simulink model "structure_contact"  (R2026b)
settings: Solver=VariableStepAuto
undefined symbols (not defined in the file or in its folder): P
libraries: sharedutil x1
settings Model: Creator=aomar  LastModifiedBy=aomar

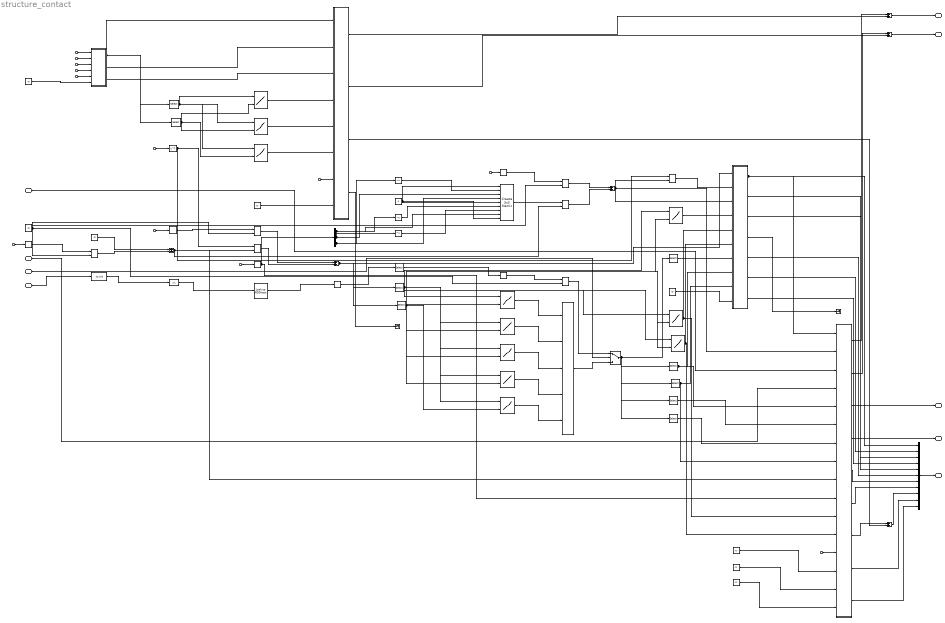
== system structure_contact ==
  body_Xe : Inport  PortName=body  Element=Xe
  body_Xe_2 : Inport  PortName=body  Element=Xe
  body_Vb : Inport  PortName=body  Element=Vb
  body_Vb_2 : Inport  PortName=body  Element=Vb
  body_omega : Inport  PortName=body  Element=omega
  body_omega_2 : Inport  PortName=body  Element=omega
  body_r_cg : Inport  PortName=body  Element=r_cg
  body_r_cg_2 : Inport  PortName=body  Element=r_cg
  body_DCM_be : Inport  PortName=body  Element=DCM_be
  body_DCM_be_2 : Inport  PortName=body  Element=DCM_be
  body_DCM_be_3 : Inport  PortName=body  Element=DCM_be
  body_DCM_be_4 : Inport  PortName=body  Element=DCM_be
  s : Inport  Port=2
  vB_d : Inport  Port=3
  use_soil : Inport  Port=4
  soil_id : Inport  Port=5
  C_nb : Math  Operator=transpose
  Cnb_rj : Product  Inputs=**  Multiplication=Matrix(*)
  Contact_Diag : BusCreator  Inputs=11
  E_g : Selector  NumberOfDimensions=2  InputPortWidth=3  IndexOptions=Index vector (dialog),Select all  Indices=2,1  OutputSizes=1
  E_j : Selector  NumberOfDimensions=2  InputPortWidth=3  IndexOptions=Index vector (dialog),Select all  Indices=2,1  OutputSizes=1
  F_c_sum : Sum
  H : Lookup_n-D  BreakpointsForDimension1=P.world.terrain.xE  BreakpointsForDimension2=P.world.terrain.yN  IndexSearchMethod=Evenly spaced points  Table=P.world.terrain.H  ExtrapMethod=Clip  InternalRulePriority=Speed  RndMeth=Simplest
      settings: InputPortMap=u0,u1
  H_g : Lookup_n-D  BreakpointsForDimension1=P.world.terrain.xE  BreakpointsForDimension2=P.world.terrain.yN  IndexSearchMethod=Evenly spaced points  Table=P.world.terrain.H  ExtrapMethod=Clip  InternalRulePriority=Speed  RndMeth=Simplest
      settings: InputPortMap=u0,u1
  K : Selector  NumberOfDimensions=2  InputPortWidth=3  IndexOptions=Index vector (dialog),Select all  Indices=2,1  OutputSizes=1
  K_map : Lookup_n-D  BreakpointsForDimension1=P.world.terrain.xE  BreakpointsForDimension2=P.world.terrain.yN  IndexSearchMethod=Evenly spaced points  Table=P.world.soil.K  ExtrapMethod=Clip  InternalRulePriority=Speed  RndMeth=Simplest
      settings: InputPortMap=u0,u1
  MF_A_trackContactNormal : MATLAB Function  TreatAsAtomicUnit=on
  MF_B_trackPlanarForces : MATLAB Function  TreatAsAtomicUnit=on
  MF_C1_gaugeWheelPoints : MATLAB Function  TreatAsAtomicUnit=on
  MF_C2_gaugeWheelContact : MATLAB Function  TreatAsAtomicUnit=on
  M_c_sum : Sum
  N_g : Selector  NumberOfDimensions=2  InputPortWidth=3  IndexOptions=Index vector (dialog),Select all  Indices=1,1  OutputSizes=1
  N_j : Selector  NumberOfDimensions=2  InputPortWidth=3  IndexOptions=Index vector (dialog),Select all  Indices=1,1  OutputSizes=1
  Omega_hat : sharedutil/Create 3x3 Matrix  aMode=aMode
      settings: LibrarySourceBlock=aerolibutil/Create 3x3 Matrix
  Ones : Constant  Value=ones(1,2*P.structure.track.Nc)  VectorParams1D=off
  P_diss_sum : Sum
  Pn : Sum
  Rc_R : Constant  Value=P.structure.contact.Rc_R  VectorParams1D=off
  Rcg_rep : Product  Inputs=**  Multiplication=Matrix(*)
  Rg_R : Constant  Value=P.structure.contact.gw.R  VectorParams1D=off
  Soil_col : Reshape  OutputDimensionality=Column vector (2-D)
  Soil_map : Concatenate  NumInputs=5  Mode=Multidimensional array
  Soil_props : Selector  InputPortWidth=6  IndexOptions=Index vector (dialog)  Indices=2:6  OutputSizes=1
  Soil_rep : Product  Inputs=**  Multiplication=Matrix(*)
  Soil_row : Reshape
  Soil_sw : Switch  Criteria=u2 ~= 0  SaturateOnIntegerOverflow=off  InputSameDT=off
  Soil_table : LookupNDDirect  InputsSelectThisObjectFromTable=Vector  Table=P.world.soilTable'  DiagnosticForOutOfRangeInput=None
  Term_K_trk : Terminator
  Term_N_gw : Terminator
  Vb_col : Reshape  OutputDimensionality=Column vector (2-D)
  Vb_pt : Sum
  Vb_rep : Product  Inputs=**  Multiplication=Matrix(*)
  Vn : Product  Inputs=**  Multiplication=Matrix(*)
  Wxr : Product  Inputs=**  Multiplication=Matrix(*)
  Xe_col : Reshape  OutputDimensionality=Column vector (2-D)
  Xe_rep : Product  Inputs=**  Multiplication=Matrix(*)
  Zero : Constant  Value=0  VectorParams1D=off
  dHdE : Lookup_n-D  BreakpointsForDimension1=P.world.terrain.xE  BreakpointsForDimension2=P.world.terrain.yN  IndexSearchMethod=Evenly spaced points  Table=P.world.terrain.dHdE  ExtrapMethod=Clip  InternalRulePriority=Speed  RndMeth=Simplest
      settings: InputPortMap=u0,u1
  dHdE_g : Lookup_n-D  BreakpointsForDimension1=P.world.terrain.xE  BreakpointsForDimension2=P.world.terrain.yN  IndexSearchMethod=Evenly spaced points  Table=P.world.terrain.dHdE  ExtrapMethod=Clip  InternalRulePriority=Speed  RndMeth=Simplest
      settings: InputPortMap=u0,u1
  dHdN : Lookup_n-D  BreakpointsForDimension1=P.world.terrain.xE  BreakpointsForDimension2=P.world.terrain.yN  IndexSearchMethod=Evenly spaced points  Table=P.world.terrain.dHdN  ExtrapMethod=Clip  InternalRulePriority=Speed  RndMeth=Simplest
      settings: InputPortMap=u0,u1
  dHdN_g : Lookup_n-D  BreakpointsForDimension1=P.world.terrain.xE  BreakpointsForDimension2=P.world.terrain.yN  IndexSearchMethod=Evenly spaced points  Table=P.world.terrain.dHdN  ExtrapMethod=Clip  InternalRulePriority=Speed  RndMeth=Simplest
      settings: InputPortMap=u0,u1
  fR : Selector  NumberOfDimensions=2  InputPortWidth=3  IndexOptions=Index vector (dialog),Select all  Indices=4,1  OutputSizes=1
  fRoll_map : Lookup_n-D  BreakpointsForDimension1=P.world.terrain.xE  BreakpointsForDimension2=P.world.terrain.yN  IndexSearchMethod=Evenly spaced points  Table=P.world.soil.fRoll  ExtrapMethod=Clip  InternalRulePriority=Speed  RndMeth=Simplest
      settings: InputPortMap=u0,u1
  gG : Constant  Value=P.structure.track.gG  VectorParams1D=off
  gS : Constant  Value=P.structure.track.gS  VectorParams1D=off
  kS : Selector  NumberOfDimensions=2  InputPortWidth=3  IndexOptions=Index vector (dialog),Select all  Indices=5,1  OutputSizes=1
  kScale_map : Lookup_n-D  BreakpointsForDimension1=P.world.terrain.xE  BreakpointsForDimension2=P.world.terrain.yN  IndexSearchMethod=Evenly spaced points  Table=P.world.soil.kScale  ExtrapMethod=Clip  InternalRulePriority=Speed  RndMeth=Simplest
      settings: InputPortMap=u0,u1
  muLat : Selector  NumberOfDimensions=2  InputPortWidth=3  IndexOptions=Index vector (dialog),Select all  Indices=3,1  OutputSizes=1
  muLat_map : Lookup_n-D  BreakpointsForDimension1=P.world.terrain.xE  BreakpointsForDimension2=P.world.terrain.yN  IndexSearchMethod=Evenly spaced points  Table=P.world.soil.muLat  ExtrapMethod=Clip  InternalRulePriority=Speed  RndMeth=Simplest
      settings: InputPortMap=u0,u1
  muP : Selector  NumberOfDimensions=2  InputPortWidth=3  IndexOptions=Index vector (dialog),Select all  Indices=1,1  OutputSizes=1
  muPeak_map : Lookup_n-D  BreakpointsForDimension1=P.world.terrain.xE  BreakpointsForDimension2=P.world.terrain.yN  IndexSearchMethod=Evenly spaced points  Table=P.world.soil.muPeak  ExtrapMethod=Clip  InternalRulePriority=Speed  RndMeth=Simplest
      settings: InputPortMap=u0,u1
  neg_p : UnaryMinus
  neg_q : UnaryMinus
  neg_r : UnaryMinus
  pqr : Demux  Outputs=3
  prmC : Constant  Value=[P.structure.contact.kc; P.structure.contact.cc]  VectorParams1D=off
  prmG : Constant  Value=[P.structure.contact.gw.on; P.structure.contact.gw.k; P.structure.contact.gw.c]  VectorParams1D=off
  prmT : Constant  Value=[P.structure.track.ell; P.structure.track.tau_d; P.structure.track.vEpsRR; P.structure.track.B; P.structure.track.chi_rmin]  VectorParams1D=off
  r_j : Sum  Inputs=+-
  rcg_col : Reshape  OutputDimensionality=Column vector (2-D)
  soil_dbl : DataTypeConversion  OutDataTypeStr=double  SaturateOnIntegerOverflow=off  RndMeth=Floor
  soil_idx0 : Bias  Bias=-1  SaturateOnIntegerOverflow=off
  w_col : Reshape  OutputDimensionality=Column vector (2-D)
  F_c : Outport
  M_c : Outport  Port=2
  sDot : Outport  Port=3
  Fx_pt : Outport  Port=4
  cdiag : Outport  Port=5
  wires:
  body_r_cg/1 -> rcg_col/1  "r_cg"
  Rg_R/1 -> MF_C1_gaugeWheelPoints/6(Rg)  "Rg_R"
  s/1 -> MF_B_trackPlanarForces/3(s)  "s"
  Ones/1 -> Soil_rep/2, Vb_rep/2, Rcg_rep/2, Xe_rep/2  "ones"
  rcg_col/1 -> Rcg_rep/1  "rcg_col"
  vB_d/1 -> MF_B_trackPlanarForces/4(vB)  "vB_d"
  use_soil/1 -> Soil_sw/2  "use_soil"
  soil_id/1 -> soil_dbl/1  "soil_id"
  body_Xe_2/1 -> MF_C1_gaugeWheelPoints/1(Xe)  "Xe"
  body_DCM_be_3/1 -> MF_C1_gaugeWheelPoints/2(DCM_be)  "DCM_be"
  body_Vb_2/1 -> MF_C1_gaugeWheelPoints/3(Vb)  "Vb"
  body_omega_2/1 -> MF_C1_gaugeWheelPoints/4(omega)  "omega"
  body_r_cg_2/1 -> MF_C1_gaugeWheelPoints/5(rcg)  "r_cg"
  Rc_R/1 -> r_j/1  "Rc_R"
  Rcg_rep/1 -> r_j/2  "Rcg_rep"
  MF_C1_gaugeWheelPoints/1(Pn_g) -> N_g/1, E_g/1, MF_C2_gaugeWheelContact/1(Pn_g)  "Pn_g"
  MF_C1_gaugeWheelPoints/2(Vn_g) -> MF_C2_gaugeWheelContact/2(Vn_g)  "Vn_g"
  MF_C1_gaugeWheelPoints/3(r_g) -> MF_C2_gaugeWheelContact/3(r_g)  "r_g"
  soil_dbl/1 -> soil_idx0/1  "soil_dbl"
  body_DCM_be/1 -> C_nb/1  "DCM_be"
  body_Xe/1 -> Xe_col/1  "Xe"
  r_j/1 -> MF_B_trackPlanarForces/9(Rcg), Wxr/2, Cnb_rj/2  "r_j"
  C_nb/1 -> Cnb_rj/1, Vn/1  "C_nb"
  Xe_col/1 -> Xe_rep/1  "Xe_col"
  E_g/1 -> dHdN_g/1, dHdE_g/1, H_g/1  "E_g"
  soil_idx0/1 -> Soil_table/1  "soil_index0"
  N_g/1 -> dHdN_g/2, H_g/2, dHdE_g/2  "N_g"
  body_omega/1 -> w_col/1  "omega"
  prmG/1 -> MF_C2_gaugeWheelContact/8(prmG)  "prmG"
  Xe_rep/1 -> Pn/1  "Xe_rep"
  Cnb_rj/1 -> Pn/2  "Cnb_rj"
  w_col/1 -> MF_B_trackPlanarForces/10(omega), pqr/1  "w_col"
  H_g/1 -> MF_C2_gaugeWheelContact/4(h)  "h_g"
  dHdE_g/1 -> MF_C2_gaugeWheelContact/5(hE)  "hE_g"
  dHdN_g/1 -> MF_C2_gaugeWheelContact/6(hN)  "hN_g"
  Soil_table/1 -> Soil_row/1  "soil_row"
  body_DCM_be_4/1 -> MF_C2_gaugeWheelContact/7(DCM_be)  "DCM_be"
  pqr/1 -> Omega_hat/8, neg_p/1  "p"
  pqr/2 -> Omega_hat/3, neg_q/1  "q"
  pqr/3 -> neg_r/1, Omega_hat/4  "r"
  Pn/1 -> MF_A_trackContactNormal/1(Pn), N_j/1, E_j/1  "Pn"
  Soil_row/1 -> Soil_props/1  "Soil_row"
  MF_C2_gaugeWheelContact/1(F_g) -> F_c_sum/2  "F_gw"
  MF_C2_gaugeWheelContact/2(M_g) -> M_c_sum/2  "M_gw"
  MF_C2_gaugeWheelContact/3(P_g) -> P_diss_sum/2  "P_gw"
  MF_C2_gaugeWheelContact/4(N_g) -> Term_N_gw/1  "N_gw"
  neg_r/1 -> Omega_hat/2  "neg_r"
  Zero/1 -> Omega_hat/9, Omega_hat/1, Omega_hat/5  "Zero"
  neg_p/1 -> Omega_hat/6  "neg_p"
  neg_q/1 -> Omega_hat/7  "neg_q"
  Soil_props/1 -> Soil_col/1  "soil_props5"
  E_j/1 -> kScale_map/1, fRoll_map/1, H/1, muLat_map/1, dHdN/1, K_map/1, dHdE/1, muPeak_map/1  "E_j"
  N_j/1 -> kScale_map/2, H/2, fRoll_map/2, muLat_map/2, dHdN/2, K_map/2, dHdE/2, muPeak_map/2  "N_j"
  body_Vb/1 -> Vb_col/1  "Vb"
  Vb_col/1 -> Vb_rep/1  "Vb_col"
  Soil_col/1 -> Soil_rep/1  "Soil_col"
  Omega_hat/1 -> Wxr/1  "Omega_hat"
  muPeak_map/1 -> Soil_map/1  "muPeak"
  K_map/1 -> Soil_map/2  "K"
  muLat_map/1 -> Soil_map/3  "muLat"
  fRoll_map/1 -> Soil_map/4  "fRoll"
  kScale_map/1 -> Soil_map/5  "kScale"
  Vb_rep/1 -> Vb_pt/1  "Vb_rep"
  Wxr/1 -> Vb_pt/2  "Wxr"
  Soil_rep/1 -> Soil_sw/1  "soil_ovr"
  Soil_map/1 -> Soil_sw/3  "soil_map"
  Vb_pt/1 -> MF_B_trackPlanarForces/2(Vb_pt), MF_A_trackContactNormal/3(Vb_pt), Vn/2  "Vb_pt"
  Soil_sw/1 -> kS/1, fR/1, muLat/1, K/1, muP/1  "soil_props"
  Vn/1 -> MF_A_trackContactNormal/2(Vn)  "Vn"
  prmC/1 -> MF_A_trackContactNormal/10(prmC)  "prmC"
  kS/1 -> MF_A_trackContactNormal/7(kS)  "kS"
  muP/1 -> MF_A_trackContactNormal/8(muP), MF_B_trackPlanarForces/5(muP)  "muP"
  muLat/1 -> MF_B_trackPlanarForces/6(muLat)  "muLat"
  fR/1 -> MF_B_trackPlanarForces/7(fR)  "fR"
  K/1 -> MF_A_trackContactNormal/9(K), MF_B_trackPlanarForces/8(K)  "K"
  H/1 -> MF_A_trackContactNormal/4(h)  "h"
  prmT/1 -> MF_B_trackPlanarForces/14(prmT)  "prmT"
  gS/1 -> MF_B_trackPlanarForces/15(gS)  "gS"
  gG/1 -> MF_B_trackPlanarForces/16(gG)  "gG"
  MF_A_trackContactNormal/1(N_pt) -> Contact_Diag/1, MF_B_trackPlanarForces/1(N_pt)  "N_pt"
  MF_A_trackContactNormal/2(N_trk) -> Contact_Diag/3  "N_trk"
  MF_A_trackContactNormal/3(muP_trk) -> Contact_Diag/5  "muP_trk"
  MF_A_trackContactNormal/4(K_trk) -> Term_K_trk/1  "K_trk"
  MF_A_trackContactNormal/5(vG_trk) -> Contact_Diag/6  "vG_trk"
  MF_A_trackContactNormal/6(pen_pt) -> Contact_Diag/2  "pen_pt"
  MF_A_trackContactNormal/7(sink_trk) -> Contact_Diag/4  "sink_trk"
  body_DCM_be_2/1 -> MF_B_trackPlanarForces/13(DCM_be)  "DCM_be"
  MF_B_trackPlanarForces/1(F_c) -> F_c_sum/1  "F_c_trk"
  MF_B_trackPlanarForces/2(M_c) -> M_c_sum/1  "M_c_trk"
  MF_B_trackPlanarForces/3(sDot) -> sDot/1  "sDot"
  MF_B_trackPlanarForces/4(Fx_pt) -> Fx_pt/1  "Fx_pt"
  MF_B_trackPlanarForces/5(Fy_trk) -> Contact_Diag/7  "Fy_trk"
  MF_B_trackPlanarForces/6(M_turn) -> Contact_Diag/8  "M_turn"
  MF_B_trackPlanarForces/7(P_diss) -> P_diss_sum/1  "P_diss_trk"
  MF_B_trackPlanarForces/8(chi_eff) -> Contact_Diag/10  "chi_eff"
  MF_B_trackPlanarForces/9(s_trk) -> Contact_Diag/11  "s_trk"
  F_c_sum/1 -> F_c/1  "F_c"
  M_c_sum/1 -> M_c/1  "M_c"
  P_diss_sum/1 -> Contact_Diag/9  "P_diss"
  Contact_Diag/1 -> cdiag/1  "cdiag"
  dHdE/1 -> MF_B_trackPlanarForces/11(hE), MF_A_trackContactNormal/5(hE)  "hE"
  dHdN/1 -> MF_B_trackPlanarForces/12(hN), MF_A_trackContactNormal/6(hN)  "hN"

== matlab function structure_contact/MF_B_trackPlanarForces ==
  settings: description=MF-B: isotropic 2-D shear law, rolling resistance, contact wrench (structure_planar_forces.m); prmT = [ell; tau_d; vEpsRR; B; chi_rmin], gS / gG of P.structure.track
  data: N_pt input; F_c output; Vb_pt input; s input; vB input; muP input; muLat input; fR input; K input; Rcg input; omega input; hE input; hN input; DCM_be input; prmT input; gS input; gG input; M_c output; sDot output; Fx_pt output; Fy_trk output; M_turn output; P_diss output; chi_eff output; s_trk output
function [F_c, M_c, sDot, Fx_pt, Fy_trk, M_turn, P_diss, chi_eff, s_trk] = trackPlanarForces(N_pt, Vb_pt, s, vB, muP, muLat, fR, K, Rcg, omega, hE, hN, DCM_be, prmT, gS, gG)
%#codegen
[F_c, M_c, sDot, Fx_pt, Fy_trk, M_turn, P_diss, chi_eff, s_trk] = structure_planar_forces(N_pt, Vb_pt, s, vB, muP, muLat, fR, K, Rcg, omega, hE, hN, DCM_be, struct('ell', prmT(1), 'tau_d', prmT(2), 'vEpsRR', prmT(3), 'B', prmT(4), 'chi_rmin', prmT(5), 'gS', gS, 'gG', gG));
end

% ---- verbatim copy of subsystems/structure/structure_planar_forces.m (generated by build_structure, do not edit here) ----
function [F_c, M_c, sDot, Fx_pt, Fy_trk, M_turn, P_diss, chi_eff, s_trk] = structure_planar_forces(N_pt, Vb_pt, s, vB, muP, muLat, fR, K, Rcg, omega, hE, hN, DCM_be, prm)
%STRUCTURE_PLANAR_FORCES  MF-B trackPlanarForces: per-point ISOTROPIC 2-D Dahl/Janosi shear (revision B, D39),
%   rolling resistance and the contact wrench (docs/specs/structure.md 2.5 / 2.6 / 4.2; owner structure, T03).
%#codegen
%
%   Inputs  N_pt [M x 1] normal forces (MF-A), Vb_pt [3 x M] point velocities in body axes (FRD),
%           s [2M x 1] shear states [s_x(1:M); s_y(1:M)] (Integrator, structure_track_shear),
%           vB [2 x 1] belt speeds [L; R] DELAYED by one 1 ms sample (D36 loop breaker),
%           muP, muLat, fR, K [1 x M] soil properties at the points, Rcg [3 x M] lever arms w.r.t. the CG (FRD),
%           omega [3 x 1] body rates (FRD), hE, hN [1 x M] terrain gradients at the points, DCM_be [3 x 3] NED->body,
%           prm = struct with the P.structure.track fields ell, tau_d, vEpsRR, gS, gG, B, chi_rmin (Nc = numel(N_pt)/2)
%   Per point j of track i:
%     v_slip = [v_b,i - v_x,j; -v_y,j]                       (belt minus ground)
%     ds/dt  = (v_slip - |v_slip| s)/K_j - (|v_b,i|/ell) s     (2-vector, |s| <= 1)
%     mu_j   = mu_p mu_lat |s| / sqrt((mu_lat s_x)^2 + (mu_p s_y)^2)   (friction ellipse along s; mu_p for |s| < 1e-6)
%     F_j    = sat_|.|( mu_j N_j [g(|s|) s/|s| + tau_d ds/dt], mu_j N_j ),  g = table prm.gS / prm.gG
%     F_rr,j = -f_r,j N_j tanh(v_x,j / vEpsRR)                (rolling resistance, body only)
%     F_c,j  = [F_x,j + F_rr,j; F_y,j; 0] + N_j n_j  applied at r_j, n_j = DCM_be [-hN; -hE; -1]/sqrt(1+hE^2+hN^2)
%              (normal force along the local terrain normal, expressed in body axes; T03 refinement of spec 2.6,
%              which applied it along -z_b: removes the spurious N sin(pitch) force of the static compliance pitch)
%   Outputs F_c, M_c [3 x 1] contact wrench about the CG (FRD), sDot [2M x 1], Fx_pt [M x 1] shear traction per
%           point (sum per track = sprocket belt load), Fy_trk [2 x 1] lateral shear force per track (FRD),
%           M_turn lateral-shear yaw moment sum(x_j F_y,j) (FRD z), P_diss = sum_i F_x,i v_b,i - sum_j F_c,j . v_j
%           (contact dissipation incl. shear slip, rolling resistance and normal damping), chi_eff =
%           (v_bR - v_bL)/(B r_FLU) (NaN for |r| < chi_rmin), s_trk [2 x 1] N-weighted mean s_x per track
M  = numel(N_pt);              % 2*Nc points (compile-time constant from the input dimension)
Nc = M/2;
F_pt = zeros(3, M);
sDot = zeros(2*M, 1);
Fx_pt = zeros(M, 1);
Fy_pt = zeros(M, 1);
gS = prm.gS;  gG = prm.gG;
for j = 1:M
    if j <= Nc, i = 1; else, i = 2; end
    vb  = vB(i);
    vx  = Vb_pt(1, j);  vy = Vb_pt(2, j);
    vsx = vb - vx;      vsy = -vy;
    vsn = sqrt(vsx*vsx + vsy*vsy);
    sx  = s(j);         sy = s(M + j);
    Kj  = max(K(j), 1e-6);
    rl  = abs(vb)/prm.ell;
    dsx = (vsx - vsn*sx)/Kj - rl*sx;
    dsy = (vsy - vsn*sy)/Kj - rl*sy;
    sDot(j) = dsx;  sDot(M + j) = dsy;
    sn  = sqrt(sx*sx + sy*sy);
    if sn < 1e-6
        mu = muP(j);  gx = 0;  gy = 0;
    else
        mu = muP(j)*muLat(j)*sn/sqrt((muLat(j)*sx)^2 + (muP(j)*sy)^2);
        gv = local_g(min(sn, 1), gS, gG);
        gx = gv*sx/sn;  gy = gv*sy/sn;
    end
    cap = mu*N_pt(j);
    fx  = cap*(gx + prm.tau_d*dsx);
    fy  = cap*(gy + prm.tau_d*dsy);
    fm  = sqrt(fx*fx + fy*fy);
    if fm > cap && fm > 0
        fx = fx*cap/fm;  fy = fy*cap/fm;
    end
    frr = -fR(j)*N_pt(j)*tanh(vx/prm.vEpsRR);
    nz  = 1/sqrt(1 + hE(j)^2 + hN(j)^2);
    nN  = -hN(j)*nz;  nE = -hE(j)*nz;  nD = -nz;            % upward terrain normal (NED)
    Fx_pt(j) = fx;  Fy_pt(j) = fy;
    F_pt(1, j) = fx + frr + N_pt(j)*(DCM_be(1,1)*nN + DCM_be(1,2)*nE + DCM_be(1,3)*nD);
    F_pt(2, j) = fy       + N_pt(j)*(DCM_be(2,1)*nN + DCM_be(2,2)*nE + DCM_be(2,3)*nD);
    F_pt(3, j) =            N_pt(j)*(DCM_be(3,1)*nN + DCM_be(3,2)*nE + DCM_be(3,3)*nD);
end
F_c = zeros(3, 1);  M_c = zeros(3, 1);
P_body = 0;  M_turn = 0;
Fy_trk = zeros(2, 1);  Fx_trk = zeros(2, 1);
for j = 1:M
    if j <= Nc, i = 1; else, i = 2; end
    f = F_pt(:, j);  r = Rcg(:, j);
    F_c = F_c + f;
    M_c = M_c + [r(2)*f(3) - r(3)*f(2); r(3)*f(1) - r(1)*f(3); r(1)*f(2) - r(2)*f(1)];
    P_body = P_body + f(1)*Vb_pt(1, j) + f(2)*Vb_pt(2, j) + f(3)*Vb_pt(3, j);
    M_turn = M_turn + r(1)*Fy_pt(j);
    Fy_trk(i) = Fy_trk(i) + Fy_pt(j);
    Fx_trk(i) = Fx_trk(i) + Fx_pt(j);
end
P_diss = Fx_trk(1)*vB(1) + Fx_trk(2)*vB(2) - P_body;
rF = -omega(3);                                  % yaw rate FLU (+ = left turn)
if abs(rF) < prm.chi_rmin
    chi_eff = NaN;
else
    chi_eff = (vB(2) - vB(1))/(prm.B*rF);
end
s_trk = zeros(2, 1);
for i = 1:2
    i0 = (i - 1)*Nc;
    sN = 0;  a = 0;  b = 0;
    for k = 1:Nc
        sN = sN + N_pt(i0 + k);
        a  = a + N_pt(i0 + k)*s(i0 + k);
        b  = b + s(i0 + k)/Nc;
    end
    if sN < 1
        s_trk(i) = b;
    else
        s_trk(i) = a/sN;
    end
end
end

% -------------------------------------------------------------------------------------------
function y = local_g(x, gS, gG)
% codegen-safe linear interpolation of the lumped Janosi table g(s) (same data as P.structure.track.gS/gG)
n = numel(gS);
if x <= gS(1)
    y = gG(1);
elseif x >= gS(n)
    y = gG(n);
else
    k = 1;
    while k < n - 1 && gS(k + 1) < x
        k = k + 1;
    end
    y = gG(k) + (gG(k + 1) - gG(k))*(x - gS(k))/(gS(k + 1) - gS(k));
end
end

== matlab function structure_contact/MF_A_trackContactNormal ==
  settings: description=MF-A: compliant normal contact of the 14 track points (structure_contact_normal.m); prmC = [kc; cc] of P.structure.contact
  data: Pn input; N_pt output; Vn input; Vb_pt input; h input; hE input; hN input; kS input; muP input; K input; prmC input; N_trk output; muP_trk output; K_trk output; vG_trk output; pen_pt output; sink_trk output
function [N_pt, N_trk, muP_trk, K_trk, vG_trk, pen_pt, sink_trk] = trackContactNormal(Pn, Vn, Vb_pt, h, hE, hN, kS, muP, K, prmC)
%#codegen
[N_pt, N_trk, muP_trk, K_trk, vG_trk, pen_pt, sink_trk] = structure_contact_normal(Pn, Vn, Vb_pt, h, hE, hN, kS, muP, K, struct('kc', prmC(1), 'cc', prmC(2)));
end

% ---- verbatim copy of subsystems/structure/structure_contact_normal.m (generated by build_structure, do not edit here) ----
function [N_pt, N_trk, muP_trk, K_trk, vG_trk, pen_pt, sink_trk] = structure_contact_normal(Pn, Vn, Vb_pt, h, hE, hN, kS, muP, K, prm)
%STRUCTURE_CONTACT_NORMAL  MF-A trackContactNormal: compliant normal contact of the 2 x Nc track points
%   (docs/specs/structure.md 2.4 / 4.1; owner structure, build task T03).
%#codegen
%
%   Inputs  Pn, Vn [3 x M] contact-point positions / velocities in NED (M = 2*prm.Nc, 1..Nc left, Nc+1..M right)
%           Vb_pt  [3 x M] contact-point velocities in body axes (FRD)
%           h, hE, hN, kS, muP, K [1 x M] terrain height (up), gradients dH/dE, dH/dN, stiffness scale,
%                  peak traction coefficient and shear modulus at the points (2-D Lookup Tables)
%           prm    struct with the P.structure.contact fields kc, cc (Nc = numel(h)/2 from the inputs)
%   Outputs N_pt [M x 1] normal force (>= 0), N_trk [2 x 1], muP_trk / K_trk [2 x 1] N-weighted means
%           (plain means while N_trk < 1 N), vG_trk [2 x 1] mean body-x ground speed of the track points,
%           pen_pt [M x 1] penetration (> 0 below the surface), sink_trk [2 x 1] N-weighted mean penetration
%
%   pen_j  = (D_j + h_j) n_z,  pen'_j = (vD_j + hE vE_j + hN vN_j) n_z,  n_z = 1/sqrt(1 + hE^2 + hN^2)
%   N_j    = [pen_j > 0] max(0, kc kS_j pen_j + cc sqrt(kS_j) pen'_j)
M  = numel(h);                 % 2*Nc points (compile-time constant from the input dimension)
Nc = M/2;
N_pt = zeros(M, 1);  pen_pt = zeros(M, 1);
N_trk = zeros(2, 1); muP_trk = zeros(2, 1); K_trk = zeros(2, 1); vG_trk = zeros(2, 1); sink_trk = zeros(2, 1);
for j = 1:M
    nz   = 1/sqrt(1 + hE(j)^2 + hN(j)^2);
    pen  = (Pn(3,j) + h(j))*nz;
    penD = (Vn(3,j) + hE(j)*Vn(2,j) + hN(j)*Vn(1,j))*nz;
    pen_pt(j) = pen;
    if pen > 0
        N_pt(j) = max(0, prm.kc*kS(j)*pen + prm.cc*sqrt(kS(j))*penD);
    end
end
for i = 1:2
    i0 = (i - 1)*Nc;
    sN = 0;
    for k = 1:Nc
        sN = sN + N_pt(i0 + k);
    end
    N_trk(i) = sN;
    a = 0; b = 0; c = 0; v = 0;
    for k = 1:Nc
        if sN < 1
            w = 1/Nc;
        else
            w = N_pt(i0 + k)/sN;
        end
        a = a + w*muP(i0 + k);
        b = b + w*K(i0 + k);
        c = c + w*pen_pt(i0 + k);
        v = v + Vb_pt(1, i0 + k)/Nc;
    end
    muP_trk(i) = a;  K_trk(i) = b;  sink_trk(i) = c;  vG_trk(i) = v;
end
end

== matlab function structure_contact/MF_C1_gaugeWheelPoints ==
  settings: description=MF-C1: positions / velocities of the mower gauge-wheel contact points (structure_gauge_points.m); Rg = P.structure.contact.gw.R
  data: Xe input; Pn_g output; DCM_be input; Vb input; omega input; rcg input; Rg input; Vn_g output; r_g output
function [Pn_g, Vn_g, r_g] = gaugeWheelPoints(Xe, DCM_be, Vb, omega, rcg, Rg)
%#codegen
[Pn_g, Vn_g, r_g] = structure_gauge_points(Xe, DCM_be, Vb, omega, rcg, Rg);
end

% ---- verbatim copy of subsystems/structure/structure_gauge_points.m (generated by build_structure, do not edit here) ----
function [Pn, Vn, r] = structure_gauge_points(Xe, DCM_be, Vb, omega, rcg, Rg)
%STRUCTURE_GAUGE_POINTS  MF-C1 gaugeWheelPoints: positions and velocities of the mower gauge-wheel contact points
%   (rigid deck on caster gauge wheels that touch the ground, the user 2026-11-15; owner structure, build task T03).
%#codegen
%
%   Inputs  Xe [3] CG position NED, DCM_be [3 x 3] NED -> body, Vb [3] CG velocity (FRD), omega [3] body rates
%           (FRD), rcg [3] CG w.r.t. R (FRD), Rg [3 x G] wheel contact points w.r.t. R (FRD, P.structure.contact.gw.R)
%   Outputs Pn, Vn [3 x G] point positions / velocities in NED, r [3 x G] lever arms w.r.t. the CG (FRD)
%
%   r_g = Rg_g - rcg,  Pn_g = Xe + C_nb r_g,  Vn_g = C_nb (Vb + omega x r_g),  C_nb = DCM_be'
%   (as the track points of structure_contact)
G  = size(Rg, 2);
Pn = zeros(3, G);  Vn = zeros(3, G);  r = zeros(3, G);
C_nb = DCM_be.';
for k = 1:G
    rk = [Rg(1, k) - rcg(1); Rg(2, k) - rcg(2); Rg(3, k) - rcg(3)];
    vb = [Vb(1) + omega(2)*rk(3) - omega(3)*rk(2); ...
          Vb(2) + omega(3)*rk(1) - omega(1)*rk(3); ...
          Vb(3) + omega(1)*rk(2) - omega(2)*rk(1)];
    r(:, k)  = rk;
    Pn(:, k) = [Xe(1); Xe(2); Xe(3)] + C_nb*rk;
    Vn(:, k) = C_nb*vb;
end
end

== matlab function structure_contact/MF_C2_gaugeWheelContact ==
  settings: description=MF-C2: compliant normal contact of the mower gauge wheels (structure_gauge_contact.m); prmG = [on; k; c] of P.structure.contact.gw
  data: Pn_g input; F_g output; Vn_g input; r_g input; h input; hE input; hN input; DCM_be input; prmG input; M_g output; P_g output; N_g output
function [F_g, M_g, P_g, N_g] = gaugeWheelContact(Pn_g, Vn_g, r_g, h, hE, hN, DCM_be, prmG)
%#codegen
[F_g, M_g, P_g, N_g] = structure_gauge_contact(Pn_g, Vn_g, r_g, h, hE, hN, DCM_be, prmG);
end

% ---- verbatim copy of subsystems/structure/structure_gauge_contact.m (generated by build_structure, do not edit here) ----
function [F_g, M_g, P_g, N_g] = structure_gauge_contact(Pn, Vn, r, h, hE, hN, DCM_be, prm)
%STRUCTURE_GAUGE_CONTACT  MF-C2 gaugeWheelContact: compliant normal contact of the mower gauge wheels
%   (rigid deck on caster gauge wheels that touch the ground, the user 2026-11-15; owner structure, build task T03).
%#codegen
%
%   Inputs  Pn, Vn [3 x G] wheel contact-point positions / velocities in NED (MF-C1 gaugeWheelPoints),
%           r [3 x G] lever arms w.r.t. the CG (FRD), h, hE, hN [1 x G] terrain height (up) and gradients dH/dE,
%           dH/dN at the points (2-D Lookup Tables), DCM_be [3 x 3] NED -> body,
%           prm = [on; k; c] of P.structure.contact.gw (on = 1 with the mower fitted, else 0; k, c per wheel)
%   Outputs F_g, M_g [3] contact wrench about the CG (FRD), P_g = -sum_g F_g . v_g (power the wheels take from the
%           body, added to the contact dissipation P_diss of Bus_StructureDiag, D40), N_g [G] normal loads (>= 0)
%
%   Per wheel (the normal law of the track points, MF-A, without the soil stiffness scale):
%     pen = (D + h) n_z,  pen' = (vD + hE vE + hN vN) n_z,  n_z = 1/sqrt(1 + hE^2 + hN^2)
%     N   = on [pen > 0] max(0, k pen + c pen'),  F = N n  along the upward terrain normal n (as MF-B)
%   No tangential force: the wheels are casters; their rolling drag stays in the mower wrench (structure_impl_mower).
G   = size(Pn, 2);
F_g = zeros(3, 1);  M_g = zeros(3, 1);  P_g = 0;  N_g = zeros(G, 1);
for k = 1:G
    nz   = 1/sqrt(1 + hE(k)^2 + hN(k)^2);
    pen  = (Pn(3, k) + h(k))*nz;
    penD = (Vn(3, k) + hE(k)*Vn(2, k) + hN(k)*Vn(1, k))*nz;
    Nk = 0;
    if pen > 0
        Nk = prm(1)*max(0, prm(2)*pen + prm(3)*penD);
    end
    N_g(k) = Nk;
    nN = -hN(k)*nz;  nE = -hE(k)*nz;  nD = -nz;            % upward terrain normal (NED)
    f  = Nk*[DCM_be(1,1)*nN + DCM_be(1,2)*nE + DCM_be(1,3)*nD; ...   % body axes (FRD), as MF-B
             DCM_be(2,1)*nN + DCM_be(2,2)*nE + DCM_be(2,3)*nD; ...
             DCM_be(3,1)*nN + DCM_be(3,2)*nE + DCM_be(3,3)*nD];
    rk = r(:, k);
    F_g = F_g + f;
    M_g = M_g + [rk(2)*f(3) - rk(3)*f(2); rk(3)*f(1) - rk(1)*f(3); rk(1)*f(2) - rk(2)*f(1)];
    P_g = P_g - Nk*(nN*Vn(1, k) + nE*Vn(2, k) + nD*Vn(3, k));
end
end
